simulink subsystem "pwm_publisher"  (R2026a)
settings: Solver=VariableStepAuto
libraries: ros2lib x2
settings Model: Creator=vulcangrip  LastModifiedBy=kjhaydon

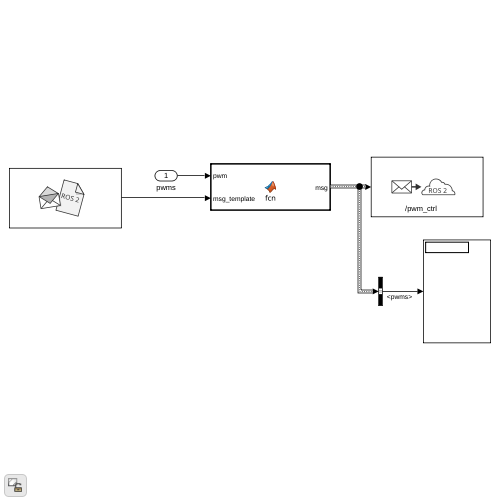
[thumbnail: Simulink's stored preview of the top-level diagram]
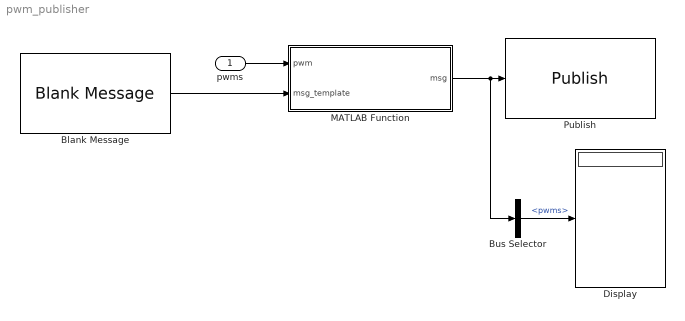
== system pwm_publisher ==
  pwms : Inport
  Blank Message : ros2lib/Blank Message  messageClass=Message  entityType=custom_interfaces/Pwms  messageType=custom_interfaces/Pwms  SampleTime=inf
  Bus Selector : BusSelector  OutputSignals=pwms
  Display : Display
  MATLAB Function : MATLAB Function  TreatAsAtomicUnit=on
  Publish : ros2lib/Publish  topicSource=Specify your own  topic=/pwm_ctrl  messageType=custom_interfaces/Pwms  QOSHistory=Keep last  QOSDepth=10  QOSReliability=Reliable  QOSDurability=Volatile  QOSDeadline=Inf  QOSLifespan=Inf  QOSLiveliness=Automatic  QOSLeaseDuration=Inf  QOSAvoidROSNamespaceConventions=off
  wires:
  pwms/1 -> MATLAB Function/1(pwm)
  Blank Message/1 -> MATLAB Function/2(msg_template)
  MATLAB Function/1(msg) -> Publish/1, Bus Selector/1
  Bus Selector/1 -> Display/1  "<pwms>"

== matlab function pwm_publisher/MATLAB Function ==
  data: pwm input; msg output Bus: SL_Bus_custom_interfaces_Pwms; msg_template input Bus: SL_Bus_custom_interfaces_Pwms
function msg = fcn(pwm, msg_template)

msg = msg_template;
msg.pwms = int32(pwm);
